simulink model "SZ08_MRR"  (R2026a)
settings: Solver=VariableStepAuto  StopTime=10  MaxStep=tau/25
InitFcn:
  | % Rendszerparaméterek
  | K = 1;
  | tau = 1;
  | xi = 1;
  | 
  | % Kezdeti értékek
  | y_0 = 0;
  | z_0 = 0;
settings Model: Creator=Szalay  LastModifiedBy=Szalay

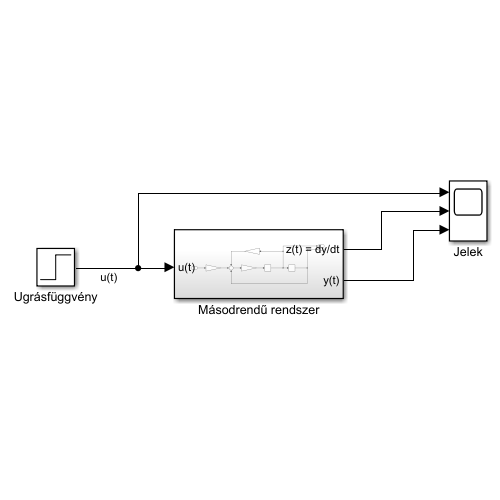
[thumbnail: Simulink's stored preview of the top-level diagram]
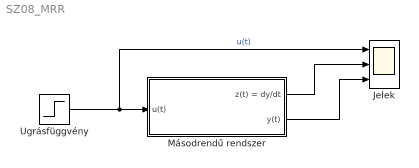
== system SZ08_MRR ==
  Jelek : Scope  NumInputPorts=3
      settings: ActiveDisplayYMinimum=-0.12499999999999997  ActiveDisplayYMaximum=1.125
  Másodrendű rendszer : Subsystem
  Ugrásfüggvény : Step  SampleTime=0
  wires:
  Ugrásfüggvény/1 -> Jelek/1, Másodrendű rendszer/1(u(t))  "u(t)"
  Másodrendű rendszer/1(z(t) = dy/dt) -> Jelek/2
  Másodrendű rendszer/2(y(t)) -> Jelek/3

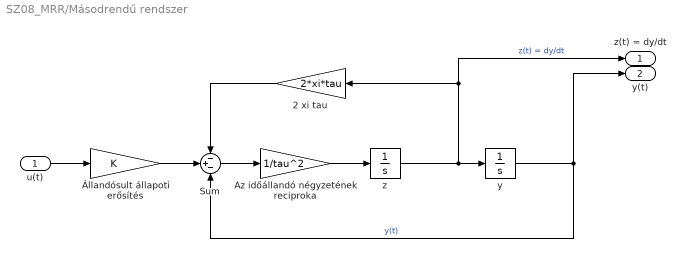
== system SZ08_MRR/Másodrendű rendszer ==
  u(t) : Inport
  2 xi tau : Gain  Gain=2*xi*tau
  Az időállandó négyzetének reciproka : Gain  Gain=1/tau^2
  Sum : Sum  Inputs=-+-
  y : Integrator  InitialCondition=y_0
  z : Integrator  InitialCondition=z_0
  Állandósult állapoti erősítés : Gain  Gain=K
  z(t) = dy/dt : Outport
  y(t) : Outport  Port=2
  wires:
  u(t)/1 -> Állandósult állapoti erősítés/1
  Állandósult állapoti erősítés/1 -> Sum/2
  z/1 -> z(t) = dy/dt/1, 2 xi tau/1, y/1  "z(t) = dy/dt"
  Az időállandó négyzetének reciproka/1 -> z/1
  Sum/1 -> Az időállandó négyzetének reciproka/1
  y/1 -> y(t)/1, Sum/3  "y(t)"
  2 xi tau/1 -> Sum/1
